simulink model "TB07_Integrated_Charging"  (R2025a)
settings: Solver=FixedStepDiscrete  StartTime=0  StopTime=TB.t_end  FixedStep=TB.dt  RelTol=1e-3
InitFcn:
  | % 모델과 같은 폴더의 초기화 스크립트를 실행해 P(설계 파라미터)와 TB(시험 조건)를 만든다.
  | run(fullfile(fileparts(get_param(bdroot, 'FileName')), 'TB07_init.m'));
values from neighbouring files (symbols this model uses):
  TB = struct()    [TB07_init.m]
libraries: fl_lib x207, nesl_utility x86
(part 1 of 5)
settings Model: Creator=hj000  LastModifiedBy=hj000
settings DataIOCC: SaveOutput=off  SignalLogging=off  SaveTime=off

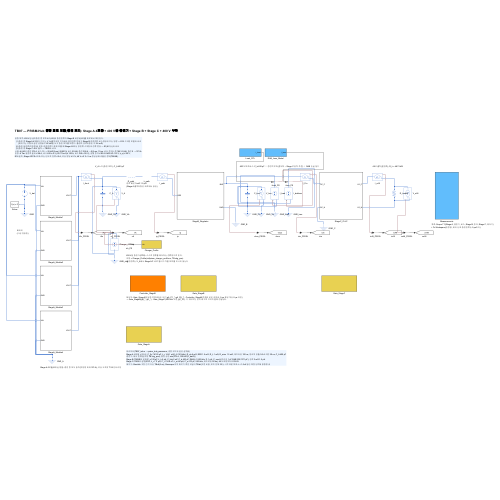
[thumbnail: Simulink's stored preview of the top-level diagram]
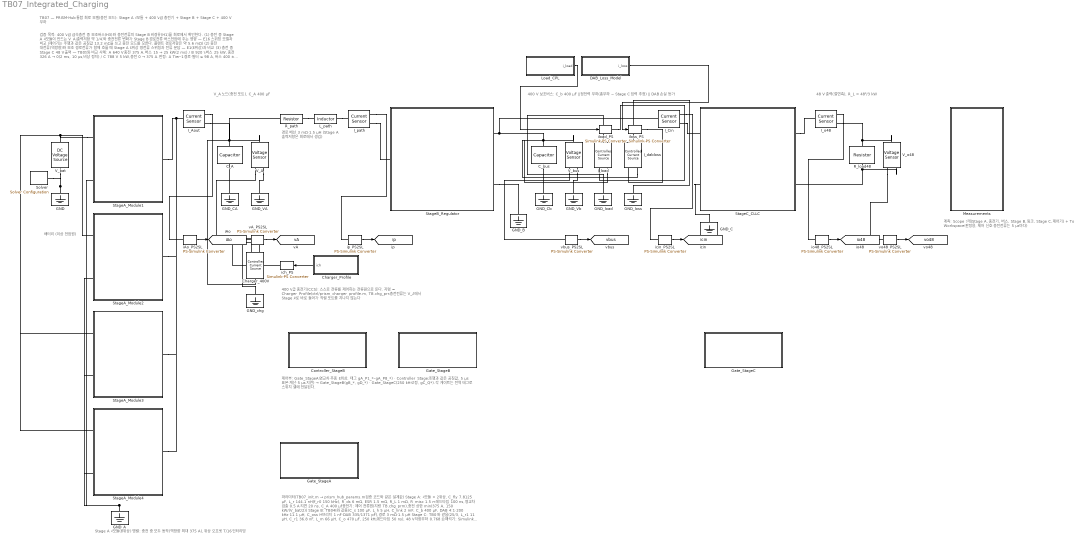
== system TB07_Integrated_Charging ==
  note: TB07 — PRISM-Hub 통합 회로 모델(충전 모드): Stage A 4모듈 + 400 V급 충전기 + Stage B + Stage C + 400 V 부하
  note: 검증 목적: 400 V급 급속충전 중 보조버스(H3)와 충전전류의 Stage B 비경유(H1)를 회로에서 확인한다.
      |   (1) 충전 중 Stage A 4모듈이 만드는 V_A(출력저항 약 1/4)와 충전전류 변화가 Stage B 경로전류·버스전압에 주는 영향 — E16 스위칭 모델과 비교
      |       (제어기는 주행과 같은 공칭값 13.2 mΩ을 쓰고 충전 모드를 모른다. 플랜트 경로저항은 약 5.6 mΩ)
      |   (2) 충전 대전류(역방향)와 보조 경로전류가 함께 흐를 때 Stage A 8위상 영전류 스위칭과 전류 분담 — E1(8위상)과 비교
      |   (3) 충전 중 Stage C 48 V 출력 — TB05와 비교
      | 사례: A 640 V 충전 375 A, 버스 15 → 25 kW(2 ms) / B 920 V 버스 25 kW, 충전 326 A → 0(2 ms, 10 µs, 비상 정지) / C 788 V 5 kW, 충전 0 → 375 A.
      | 판정: A Tier-1(경로·필터 ≤ 98 A, 버스 400 ± 8 V), B·C Tier-2(≤ 100 A, 버스 384–416 V), 공통 링크 ≤ 80 A·8 kW·90–110 V, |v_s| ≤ 90 V,
      | E16 일치, Stage A ZCS ≤ 5 % 또는 턴오프 전류 ≤ 2 A, 위상 분담 ≤ 5 %, 48 V ± 2 %. 5 ns 정상상태 리플은 정보(TB04B).
  note: 배터리
      | (이상 전압원)
  note: V_A 노드(충전 포트), C_A 400 µF
  note: 400 V급 충전기(CCS): 스스로 전류를 제어하는 전류원으로 둔다.
      | 지령 = Charger_Profile(ctrl/prism_charger_profile.m, TB.chg_prm)
      | 충전전류는 V_A에서 Stage A로 바로 들어가 직렬 포트를 지나지 않는다
  note: Stage A 4모듈(8위상) 병렬: 충전 중 모두 동작(역방향 최대 375 A), 위상 오프셋 T/16 인터리빙
  note: 경로 배선 3 mΩ·1.5 µH
      | (Stage A 출력저항은 회로에서 생김)
  note: 400 V 보조버스: C_b 400 µF ∥ 정전력 부하(총부하 − Stage C 입력 추정) ∥ DAB 손실 등가
  note: 48 V 출력(절연측), R_L = 48²/3 kW
  note: 제어부: Gate_StageA(영교차 추종 8위상, 태그 gA_P1_*–gA_P8_*) · Controller_StageB(주행과 같은 공칭값, 5 µs 표본·계산·5 µs 지연)
      | → Gate_StageB(gB_*, gD_*) · Gate_StageC(250 kHz 고정, gC_Q*). 각 게이트는 전역 태그로 스위치 셀에 전달된다.
  note: 계측: Scope 7개(Stage A, 충전기, 버스, Stage B, 링크, Stage C, 제어기)
      | + To Workspace(판정용, 제어 신호·충전전류는 5 µs마다)
  note: 파라미터(TB07_init.m → prism_hub_params.m, 검증 코드와 같은 설계값)
      | Stage A: 4모듈 × 2위상, C_fly 7.8125 µF, L_r 144.1 nH(f_r0 150 kHz), R_ds 6 mΩ, ESR 1.5 mΩ, R_L 1 mΩ, R_misc 1.5 mΩ, 데드타임 100 ns, 영교차 검출 0.5 A·지연 20 ns, C_A 400 µF
      | 충전기: 제어 전류원(지령 TB.chg_prm), 충전 상한 min(375 A, 150 kW/(V_bat/2))
      | Stage B: TB04B와 같음(C_s 100 µF, L_h 5 µH, C_link 2 mF, C_b 400 µF, DAB 4:1·200 kHz·11.1 µH, C_oss H-브리지 1 nF·DAB 335/1371 pF), 경로 3 mΩ·1.5 µH
      | Stage C: TB05와 같음(25/3, L_r1 11 µH, C_r1 36.8 nF, L_m 66 µH, C_o 470 µF, 250 kHz, 데드타임 50 ns), 48 V 저항부하 0.768 Ω
      | 해석기: Simulink 고정 간격 이산 TB.dt(5 ns), Simscape 지역 해석기 후진 오일러 TB.dt(고정 비용, 모드 반복 3회). 시작 표본 보호: t < 1.5 dt 동안 측정 입력에 평형점 값
  C_A : fl_lib/Electrical/Electrical Elements/Capacitor  c=TB.A.CA F  r=1e-6 Ohm  g=0 1/Ohm  i_specify=off  i_priority=None  i=0 A  i_nominal_specify=off  i_nominal_value=1  i_nominal_unit=A  v_specify=off  v_priority=None  v=0 V  v_nominal_specify=off  v_nominal_value=1  v_nominal_unit=V  vc_specify=on  vc_priority=High  vc=TB.vA0 V  vc_nominal_specify=off  vc_nominal_value=1  vc_nominal_unit=V
  C_bus : fl_lib/Electrical/Electrical Elements/Capacitor  c=TB.Cb F  r=1e-6 Ohm  g=0 1/Ohm  i_specify=off  i_priority=None  i=0 A  i_nominal_specify=off  i_nominal_value=1  i_nominal_unit=A  v_specify=off  v_priority=None  v=0 V  v_nominal_specify=off  v_nominal_value=1  v_nominal_unit=V  vc_specify=on  vc_priority=High  vc=TB.vb0 V  vc_nominal_specify=off  vc_nominal_value=1  vc_nominal_unit=V
  Charger_400V : fl_lib/Electrical/Electrical Sources/Controlled Current Source
  Charger_Profile : Subsystem
  Controller_StageB : Subsystem
  DAB_Loss_Model : Subsystem
  GND : fl_lib/Electrical/Electrical Elements/Electrical Reference
  GND_A : fl_lib/Electrical/Electrical Elements/Electrical Reference
  GND_B : fl_lib/Electrical/Electrical Elements/Electrical Reference
  GND_C : fl_lib/Electrical/Electrical Elements/Electrical Reference
  GND_CA : fl_lib/Electrical/Electrical Elements/Electrical Reference
  GND_Cb : fl_lib/Electrical/Electrical Elements/Electrical Reference
  GND_VA : fl_lib/Electrical/Electrical Elements/Electrical Reference
  GND_Vb : fl_lib/Electrical/Electrical Elements/Electrical Reference
  GND_chg : fl_lib/Electrical/Electrical Elements/Electrical Reference
  GND_load : fl_lib/Electrical/Electrical Elements/Electrical Reference
  GND_loss : fl_lib/Electrical/Electrical Elements/Electrical Reference
  Gate_StageA : Subsystem
  Gate_StageB : Subsystem
  Gate_StageC : Subsystem
  I_Aout : fl_lib/Electrical/Electrical Sensors/Current Sensor
  I_Cin : fl_lib/Electrical/Electrical Sensors/Current Sensor
  I_dabloss : fl_lib/Electrical/Electrical Sources/Controlled Current Source
  I_load : fl_lib/Electrical/Electrical Sources/Controlled Current Source
  I_o48 : fl_lib/Electrical/Electrical Sensors/Current Sensor
  I_path : fl_lib/Electrical/Electrical Sensors/Current Sensor
  L_path : fl_lib/Electrical/Electrical Elements/Inductor  l=TB.Lpath H  r=0 Ohm  g=1e-9 1/Ohm  i_specify=off  i_priority=None  i=0 A  i_nominal_specify=off  i_nominal_value=1  i_nominal_unit=A  v_specify=off  v_priority=None  v=0 V  v_nominal_specify=off  v_nominal_value=1  v_nominal_unit=V  i_L_specify=on  i_L_priority=High  i_L=TB.ip0 A  i_L_nominal_specify=off  i_L_nominal_value=1  i_L_nominal_unit=A
  Load_CPL : Subsystem
  Measurements : Subsystem
  R_load48 : fl_lib/Electrical/Electrical Elements/Resistor  R=TB.RL_C Ohm  i_specify=off  i_priority=None  i=0 A  i_nominal_specify=off  i_nominal_value=1  i_nominal_unit=A  v_specify=off  v_priority=None  v=0 V  v_nominal_specify=off  v_nominal_value=1  v_nominal_unit=V
  R_path : fl_lib/Electrical/Electrical Elements/Resistor  R=TB.Rpath Ohm  i_specify=off  i_priority=None  i=0 A  i_nominal_specify=off  i_nominal_value=1  i_nominal_unit=A  v_specify=off  v_priority=None  v=0 V  v_nominal_specify=off  v_nominal_value=1  v_nominal_unit=V
  Solver : nesl_utility/Solver Configuration  PhysicalDomain=network_engine_domain  SubClassName=solver  LeftPortType=input  RightPortType=generic  Tones=[]  Harmonics=[]  SimulateNoise=off  Profile=off  UseLocalSampling=off  EnableSwitchedLinearOptims=on  FrequencyDomain=off  UseCCode=off  RelTol=0.001  AbsTol=0.001  MinStep=1e-09  ToWorkspace=off  RevertToSquareIcSolve=off  NumHomotopyIterations=100  PhasorMode=off  PhasorModeNumHarmonics=1  ConsistencySolver=NEWTON_XTOL_AFTER_FTOL  IndexReductionMethod=DerivativeReplacement  DoDC=off  ResidualTolerance=1e-9  ConsistencyTolSource=GLOBAL  ConsistencyAbsTol=0.001  ConsistencyRelTol=0.001  ConsistencyTolFactor=0.001  UseLocalSolver=on  LocalSolverChoice=NE_BACKWARD_EULER_ADVANCER  ResolveIndetEquations=on  FunctionEvalNumThread=1  LocalSolverSampleTime=TB.dt  DoFixedCost=on  MaxNonlinIter=3  MaxModeIter=2  ComputeImpulses=off  ImpulseIterations=2  LinearAlgebra=auto  LinearAlgebraNumThread=0  EquationFormulation=NE_TIME_EF  DelaysMemoryBudget=1024  AutomaticFiltering=on  FilteringTimeConstant=0.001  PartitionStorageMethod=AS_NEEDED  PartitionMemoryBudget=1024  PartitionMethod=ROBUST  MultibodyUseLocalSolver=off  MultibodyLocalSolverChoice=ODE1  MultibodyLocalSolverSampleTime=0.001
  StageA_Module1 : Subsystem
  StageA_Module2 : Subsystem
  StageA_Module3 : Subsystem
  StageA_Module4 : Subsystem
  StageB_Regulator : Subsystem
  StageC_CLLC : Subsystem
  V_A : fl_lib/Electrical/Electrical Sensors/Voltage Sensor
  V_bat : fl_lib/Electrical/Electrical Sources/DC Voltage Source  v0=TB.vbat V
  V_bus : fl_lib/Electrical/Electrical Sensors/Voltage Sensor
  V_o48 : fl_lib/Electrical/Electrical Sensors/Voltage Sensor
  iAo_PS2SL : nesl_utility/PS-Simulink Converter  PhysicalDomain=network_engine_domain  SubClassName=ps_output  LeftPortType=input  RightPortType=output  PseudoPeriodic=off  Frequencies=[]  VectorFormat=inherit  Unit=inherit  AffineConversion=off
  ich_PS : nesl_utility/Simulink-PS Converter  PhysicalDomain=network_engine_domain  SubClassName=ps_input  LeftPortType=input  RightPortType=output  PseudoPeriodic=off  Frequencies=[]  NoiseDistribution=none  NoiseParameters=[]  Unit=1  AffineConversion=off  FilteringAndDerivatives=provide  SimscapeFilterOrder=1  InputFilterTimeConstant=0.001  UdotUserProvided=0
  icin_PS2SL : nesl_utility/PS-Simulink Converter  PhysicalDomain=network_engine_domain  SubClassName=ps_output  LeftPortType=input  RightPortType=output  PseudoPeriodic=off  Frequencies=[]  VectorFormat=inherit  Unit=inherit  AffineConversion=off
  iload_PS : nesl_utility/Simulink-PS Converter  PhysicalDomain=network_engine_domain  SubClassName=ps_input  LeftPortType=input  RightPortType=output  PseudoPeriodic=off  Frequencies=[]  NoiseDistribution=none  NoiseParameters=[]  Unit=1  AffineConversion=off  FilteringAndDerivatives=provide  SimscapeFilterOrder=1  InputFilterTimeConstant=0.001  UdotUserProvided=0
  iloss_PS : nesl_utility/Simulink-PS Converter  PhysicalDomain=network_engine_domain  SubClassName=ps_input  LeftPortType=input  RightPortType=output  PseudoPeriodic=off  Frequencies=[]  NoiseDistribution=none  NoiseParameters=[]  Unit=1  AffineConversion=off  FilteringAndDerivatives=provide  SimscapeFilterOrder=1  InputFilterTimeConstant=0.001  UdotUserProvided=0
  io48_PS2SL : nesl_utility/PS-Simulink Converter  PhysicalDomain=network_engine_domain  SubClassName=ps_output  LeftPortType=input  RightPortType=output  PseudoPeriodic=off  Frequencies=[]  VectorFormat=inherit  Unit=inherit  AffineConversion=off
  ip_PS2SL : nesl_utility/PS-Simulink Converter  PhysicalDomain=network_engine_domain  SubClassName=ps_output  LeftPortType=input  RightPortType=output  PseudoPeriodic=off  Frequencies=[]  VectorFormat=inherit  Unit=inherit  AffineConversion=off
  vA_PS2SL : nesl_utility/PS-Simulink Converter  PhysicalDomain=network_engine_domain  SubClassName=ps_output  LeftPortType=input  RightPortType=output  PseudoPeriodic=off  Frequencies=[]  VectorFormat=inherit  Unit=inherit  AffineConversion=off
  vbus_PS2SL : nesl_utility/PS-Simulink Converter  PhysicalDomain=network_engine_domain  SubClassName=ps_output  LeftPortType=input  RightPortType=output  PseudoPeriodic=off  Frequencies=[]  VectorFormat=inherit  Unit=inherit  AffineConversion=off
  vo48_PS2SL : nesl_utility/PS-Simulink Converter  PhysicalDomain=network_engine_domain  SubClassName=ps_output  LeftPortType=input  RightPortType=output  PseudoPeriodic=off  Frequencies=[]  VectorFormat=inherit  Unit=inherit  AffineConversion=off
  tag scope: iAo=global, icin=global, io48=global, ip=global, vA=global, vbus=global, vo48=global
  wires:
  iAo_PS2SL/1 -> [iAo]
  vA_PS2SL/1 -> [vA]
  ip_PS2SL/1 -> [ip]
  vbus_PS2SL/1 -> [vbus]
  icin_PS2SL/1 -> [icin]
  io48_PS2SL/1 -> [io48]
  vo48_PS2SL/1 -> [vo48]
  Load_CPL/1(i_load) -> iload_PS/1
  DAB_Loss_Model/1(i_loss) -> iloss_PS/1
  Charger_Profile/1(ich) -> ich_PS/1
  connections:
  GND/LConn1 -- Solver/RConn1 -- V_bat/RConn1
  StageA_Module1/LConn1 -- V_bat/LConn1 -- StageA_Module2/LConn1 -- StageA_Module3/LConn1 -- StageA_Module4/LConn1
  StageA_Module1/LConn2 -- StageA_Module2/LConn2 -- StageA_Module3/LConn2 -- GND_A/LConn1 -- StageA_Module4/LConn2
  StageA_Module1/RConn1 -- StageA_Module2/RConn1 -- StageA_Module3/RConn1 -- I_Aout/LConn1 -- StageA_Module4/RConn1
  I_Aout/RConn2 -- V_A/LConn1 -- Charger_400V/LConn1 -- C_A/LConn1 -- R_path/LConn1
  C_A/RConn1 -- GND_CA/LConn1
  V_A/RConn2 -- GND_VA/LConn1
  Charger_400V/RConn2 -- GND_chg/LConn1
  ich_PS/RConn1 -- Charger_400V/RConn1
  R_path/RConn1 -- L_path/LConn1
  L_path/RConn1 -- I_path/LConn1
  I_path/RConn2 -- StageB_Regulator/LConn1
  StageB_Regulator/RConn1 -- I_Cin/LConn1 -- V_bus/LConn1 -- I_load/RConn2 -- C_bus/LConn1 -- I_dabloss/RConn2
  StageB_Regulator/RConn2 -- GND_B/LConn1
  C_bus/RConn1 -- GND_Cb/LConn1
  V_bus/RConn2 -- GND_Vb/LConn1
  I_load/LConn1 -- GND_load/LConn1
  I_dabloss/LConn1 -- GND_loss/LConn1
  iload_PS/RConn1 -- I_load/RConn1
  iloss_PS/RConn1 -- I_dabloss/RConn1
  I_Cin/RConn2 -- StageC_CLLC/LConn1
  StageC_CLLC/LConn2 -- GND_C/LConn1
  StageC_CLLC/RConn1 -- I_o48/LConn1
  R_load48/LConn1 -- I_o48/RConn2 -- V_o48/LConn1
  StageC_CLLC/RConn2 -- R_load48/RConn1 -- V_o48/RConn2
  I_Aout/RConn1 -- iAo_PS2SL/LConn1
  V_A/RConn1 -- vA_PS2SL/LConn1
  I_path/RConn1 -- ip_PS2SL/LConn1
  V_bus/RConn1 -- vbus_PS2SL/LConn1
  I_Cin/RConn1 -- icin_PS2SL/LConn1
  I_o48/RConn1 -- io48_PS2SL/LConn1
  V_o48/RConn1 -- vo48_PS2SL/LConn1

== system TB07_Integrated_Charging/Charger_Profile ==
  note: 충전기 출력전류 지령 [i0 i1 t_sw t_ramp]: t_sw부터 t_ramp 동안 i0 → i1 선형
  Charger_Current : MATLAB Function  TreatAsAtomicUnit=on
  Clock : DigitalClock  SampleTime=TB.dt
  chg_prm : Constant  Value=TB.chg_prm
  ich : Outport
  tag scope: ich=global
  wires:
  Clock/1 -> Charger_Current/1(t)
  chg_prm/1 -> Charger_Current/2(prm)
  Charger_Current/1(ich) -> ich/1, [ich]

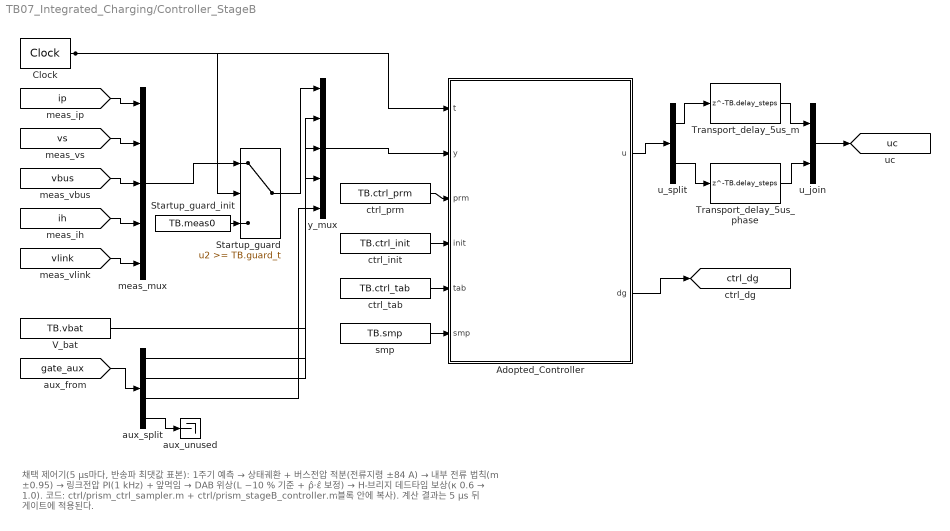
== system TB07_Integrated_Charging/Controller_StageB ==
  note: 채택 제어기(5 µs마다, 반송파 최댓값 표본): 1주기 예측 → 상태궤환 + 버스전압 적분(전류지령 ±84 A) → 내부 전류 법칙(m ±0.95)
      | → 링크전압 PI(1 kHz) + 앞먹임 → DAB 위상(L −10 % 기준 + ρ̂·ε̂ 보정) → H-브리지 데드타임 보상(κ 0.6 → 1.0).
      | 코드: ctrl/prism_ctrl_sampler.m + ctrl/prism_stageB_controller.m(블록 안에 복사). 계산 결과는 5 µs 뒤 게이트에 적용된다.
  Adopted_Controller : MATLAB Function  TreatAsAtomicUnit=on
  Clock : DigitalClock  SampleTime=TB.dt
  Startup_guard : Switch  Threshold=TB.guard_t  SaturateOnIntegerOverflow=off  InputSameDT=off
  Startup_guard_init : Constant  Value=TB.meas0
  Transport_delay_5us_m : Delay  DelayLength=TB.delay_steps  InitialCondition=TB.uc0(1)
  Transport_delay_5us_phase : Delay  DelayLength=TB.delay_steps  InitialCondition=TB.uc0(2)
  V_bat : Constant  Value=TB.vbat
  aux_split : Demux  Outputs=[1 1 1 3]
  aux_unused : Terminator
  ctrl_init : Constant  Value=TB.ctrl_init
  ctrl_prm : Constant  Value=TB.ctrl_prm
  ctrl_tab : Constant  Value=TB.ctrl_tab
  meas_mux : Mux  Inputs=5
  smp : Constant  Value=TB.smp
  u_join : Mux  Inputs=2
  u_split : Demux  Outputs=2
  y_mux : Mux  Inputs=5
  tag scope: ctrl_dg=global, uc=global
  wires:
  [ip] -> meas_mux/1
  [vs] -> meas_mux/2
  [vbus] -> meas_mux/3
  [ih] -> meas_mux/4
  [vlink] -> meas_mux/5
  Startup_guard_init/1 -> Startup_guard/3
  meas_mux/1 -> Startup_guard/1
  Clock/1 -> Startup_guard/2, Adopted_Controller/1(t)
  Startup_guard/1 -> y_mux/1
  V_bat/1 -> y_mux/2
  [gate_aux] -> aux_split/1
  aux_split/1 -> y_mux/3
  aux_split/2 -> y_mux/4
  aux_split/3 -> y_mux/5
  aux_split/4 -> aux_unused/1
  y_mux/1 -> Adopted_Controller/2(y)
  ctrl_prm/1 -> Adopted_Controller/3(prm)
  ctrl_init/1 -> Adopted_Controller/4(init)
  ctrl_tab/1 -> Adopted_Controller/5(tab)
  smp/1 -> Adopted_Controller/6(smp)
  Adopted_Controller/1(u) -> u_split/1
  u_split/1 -> Transport_delay_5us_m/1
  u_split/2 -> Transport_delay_5us_phase/1
  Transport_delay_5us_m/1 -> u_join/1
  Transport_delay_5us_phase/1 -> u_join/2
  u_join/1 -> [uc]
  Adopted_Controller/2(dg) -> [ctrl_dg]

== system TB07_Integrated_Charging/DAB_Loss_Model ==
  note: DAB 손실 등가: 직전 주기 평균 링크전력 p̄로 P_loss = (1/η − 1)max(p̄,0) + (1 − η)max(−p̄,0) − R_dab·mean(i_L²)
      | (η = 0.96, 검증 모델과 같음)을 버스 전류 P_loss/v_bus로 끈다. 회로의 R_dab 손실은 빼서 중복을 막는다.
  Clock : DigitalClock  SampleTime=TB.dt
  DAB_Loss : MATLAB Function  TreatAsAtomicUnit=on
  Startup_guard : Switch  Threshold=TB.guard_t  SaturateOnIntegerOverflow=off  InputSameDT=off
  Startup_guard_init : Constant  Value=TB.loss_meas0
  iloss_z1 : UnitDelay  SampleTime=TB.dt  HasFrameUpgradeWarning=on
  loss_prm : Constant  Value=TB.loss_prm
  meas_mux : Mux
  meas_split : Demux
  ploss0 : Constant  Value=TB.ploss0
  i_loss : Outport
  wires:
  [vlink] -> meas_mux/1
  [ilink] -> meas_mux/2
  [iL] -> meas_mux/3
  [vbus] -> meas_mux/4
  Startup_guard_init/1 -> Startup_guard/3
  meas_mux/1 -> Startup_guard/1
  Clock/1 -> Startup_guard/2, DAB_Loss/1(t)
  Startup_guard/1 -> meas_split/1
  meas_split/1 -> DAB_Loss/2(vl)
  meas_split/2 -> DAB_Loss/3(il)
  meas_split/3 -> DAB_Loss/4(iL)
  meas_split/4 -> DAB_Loss/5(vb)
  loss_prm/1 -> DAB_Loss/6(prm)
  ploss0/1 -> DAB_Loss/7(ploss0)
  DAB_Loss/1(iloss) -> iloss_z1/1
  iloss_z1/1 -> i_loss/1

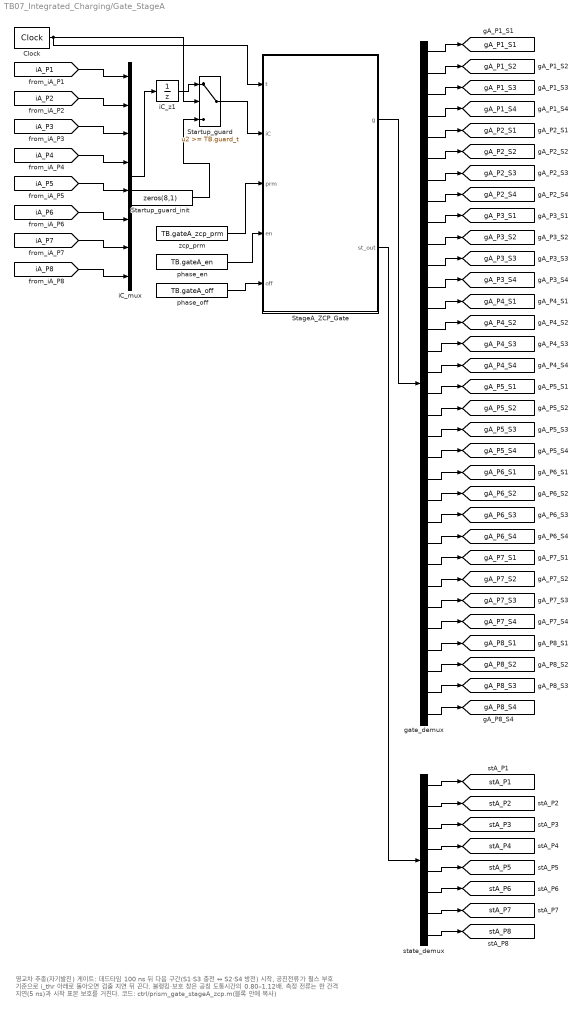
== system TB07_Integrated_Charging/Gate_StageA ==
  note: 영교차 추종(자기발진) 게이트: 데드타임 100 ns 뒤 다음 구간(S1·S3 충전 ↔ S2·S4 방전) 시작,
      | 공진전류가 펄스 부호 기준으로 i_thr 아래로 돌아오면 검출 지연 뒤 끈다. 블랭킹·보호 창은 공칭 도통시간의 0.80–1.12배.
      | 측정 전류는 한 간격 지연(5 ns)과 시작 표본 보호를 거친다. 코드: ctrl/prism_gate_stageA_zcp.m(블록 안에 복사)
  Clock : DigitalClock  SampleTime=TB.dt
  StageA_ZCP_Gate : MATLAB Function  TreatAsAtomicUnit=on
  Startup_guard : Switch  Threshold=TB.guard_t  SaturateOnIntegerOverflow=off  InputSameDT=off
  Startup_guard_init : Constant  Value=zeros(8,1)
  gate_demux : Demux  Outputs=[1 1 1 1 1 1 1 1 1 1 1 1 1 1 1 1 1 1 1 1 1 1 1 1 1 1 1 1 1 1 1 1]
  iC_mux : Mux  Inputs=8
  iC_z1 : UnitDelay  SampleTime=TB.dt  HasFrameUpgradeWarning=on
  phase_en : Constant  Value=TB.gateA_en
  phase_off : Constant  Value=TB.gateA_off
  state_demux : Demux  Outputs=[1 1 1 1 1 1 1 1]
  zcp_prm : Constant  Value=TB.gateA_zcp_prm
  tag scope: gA_P1_S1=global, gA_P1_S2=global, gA_P1_S3=global, gA_P1_S4=global, gA_P2_S1=global, gA_P2_S2=global, gA_P2_S3=global, gA_P2_S4=global, gA_P3_S1=global, gA_P3_S2=global, gA_P3_S3=global, gA_P3_S4=global, gA_P4_S1=global, gA_P4_S2=global, gA_P4_S3=global, gA_P4_S4=global, gA_P5_S1=global, gA_P5_S2=global, gA_P5_S3=global, gA_P5_S4=global, gA_P6_S1=global, gA_P6_S2=global, gA_P6_S3=global, gA_P6_S4=global, gA_P7_S1=global, gA_P7_S2=global, gA_P7_S3=global, gA_P7_S4=global, gA_P8_S1=global, gA_P8_S2=global, gA_P8_S3=global, gA_P8_S4=global, stA_P1=global, stA_P2=global, stA_P3=global, stA_P4=global, stA_P5=global, stA_P6=global, stA_P7=global, stA_P8=global
  wires:
  [iA_P1] -> iC_mux/1
  [iA_P2] -> iC_mux/2
  [iA_P3] -> iC_mux/3
  [iA_P4] -> iC_mux/4
  [iA_P5] -> iC_mux/5
  [iA_P6] -> iC_mux/6
  [iA_P7] -> iC_mux/7
  [iA_P8] -> iC_mux/8
  iC_mux/1 -> iC_z1/1
  Startup_guard_init/1 -> Startup_guard/3
  iC_z1/1 -> Startup_guard/1
  Clock/1 -> Startup_guard/2, StageA_ZCP_Gate/1(t)
  Startup_guard/1 -> StageA_ZCP_Gate/2(iC)
  zcp_prm/1 -> StageA_ZCP_Gate/3(prm)
  phase_en/1 -> StageA_ZCP_Gate/4(en)
  phase_off/1 -> StageA_ZCP_Gate/5(off)
  StageA_ZCP_Gate/1(g) -> gate_demux/1
  gate_demux/1 -> [gA_P1_S1]
  gate_demux/2 -> [gA_P1_S2]
  gate_demux/3 -> [gA_P1_S3]
  gate_demux/4 -> [gA_P1_S4]
  gate_demux/5 -> [gA_P2_S1]
  gate_demux/6 -> [gA_P2_S2]
  gate_demux/7 -> [gA_P2_S3]
  gate_demux/8 -> [gA_P2_S4]
  gate_demux/9 -> [gA_P3_S1]
  gate_demux/10 -> [gA_P3_S2]
  gate_demux/11 -> [gA_P3_S3]
  gate_demux/12 -> [gA_P3_S4]
  gate_demux/13 -> [gA_P4_S1]
  gate_demux/14 -> [gA_P4_S2]
  gate_demux/15 -> [gA_P4_S3]
  gate_demux/16 -> [gA_P4_S4]
  gate_demux/17 -> [gA_P5_S1]
  gate_demux/18 -> [gA_P5_S2]
  gate_demux/19 -> [gA_P5_S3]
  gate_demux/20 -> [gA_P5_S4]
  gate_demux/21 -> [gA_P6_S1]
  gate_demux/22 -> [gA_P6_S2]
  gate_demux/23 -> [gA_P6_S3]
  gate_demux/24 -> [gA_P6_S4]
  gate_demux/25 -> [gA_P7_S1]
  gate_demux/26 -> [gA_P7_S2]
  gate_demux/27 -> [gA_P7_S3]
  gate_demux/28 -> [gA_P7_S4]
  gate_demux/29 -> [gA_P8_S1]
  gate_demux/30 -> [gA_P8_S2]
  gate_demux/31 -> [gA_P8_S3]
  gate_demux/32 -> [gA_P8_S4]
  StageA_ZCP_Gate/2(st_out) -> state_demux/1
  state_demux/1 -> [stA_P1]
  state_demux/2 -> [stA_P2]
  state_demux/3 -> [stA_P3]
  state_demux/4 -> [stA_P4]
  state_demux/5 -> [stA_P5]
  state_demux/6 -> [stA_P6]
  state_demux/7 -> [stA_P7]
  state_demux/8 -> [stA_P8]

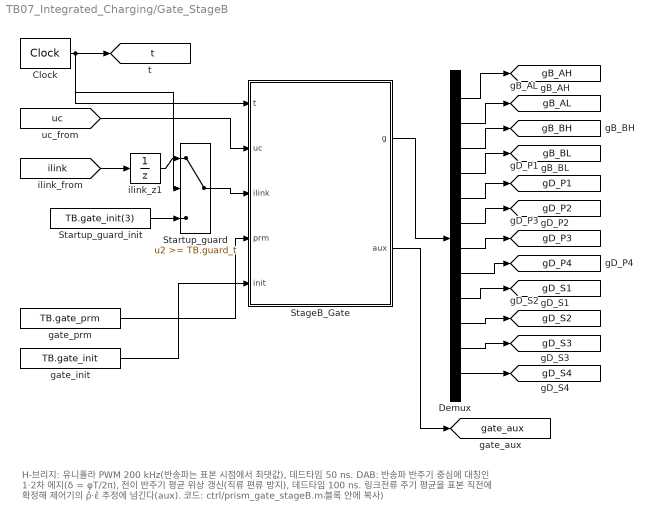
== system TB07_Integrated_Charging/Gate_StageB ==
  note: H-브리지: 유니폴라 PWM 200 kHz(반송파는 표본 시점에서 최댓값), 데드타임 50 ns.
      | DAB: 반송파 반주기 중심에 대칭인 1·2차 에지(δ = φT/2π), 전이 반주기 평균 위상 갱신(직류 편류 방지), 데드타임 100 ns.
      | 링크전류 주기 평균을 표본 직전에 확정해 제어기의 ρ̂·ε̂ 추정에 넘긴다(aux). 코드: ctrl/prism_gate_stageB.m(블록 안에 복사)
  Clock : DigitalClock  SampleTime=TB.dt
  Demux : Demux  Outputs=12
  StageB_Gate : MATLAB Function  TreatAsAtomicUnit=on
  Startup_guard : Switch  Threshold=TB.guard_t  SaturateOnIntegerOverflow=off  InputSameDT=off
  Startup_guard_init : Constant  Value=TB.gate_init(3)
  gate_init : Constant  Value=TB.gate_init
  gate_prm : Constant  Value=TB.gate_prm
  ilink_z1 : UnitDelay  SampleTime=TB.dt  HasFrameUpgradeWarning=on
  tag scope: gB_AH=global, gB_AL=global, gB_BH=global, gB_BL=global, gD_P1=global, gD_P2=global, gD_P3=global, gD_P4=global, gD_S1=global, gD_S2=global, gD_S3=global, gD_S4=global, gate_aux=global, t=global
  wires:
  Startup_guard_init/1 -> Startup_guard/3
  Clock/1 -> [t], StageB_Gate/1(t), Startup_guard/2
  [uc] -> StageB_Gate/2(uc)
  [ilink] -> ilink_z1/1
  ilink_z1/1 -> Startup_guard/1
  Startup_guard/1 -> StageB_Gate/3(ilink)
  gate_prm/1 -> StageB_Gate/4(prm)
  gate_init/1 -> StageB_Gate/5(init)
  StageB_Gate/1(g) -> Demux/1
  Demux/1 -> [gB_AH]
  Demux/2 -> [gB_AL]
  Demux/3 -> [gB_BH]
  Demux/4 -> [gB_BL]
  Demux/5 -> [gD_P1]
  Demux/6 -> [gD_P2]
  Demux/7 -> [gD_P3]
  Demux/8 -> [gD_P4]
  Demux/9 -> [gD_S1]
  Demux/10 -> [gD_S2]
  Demux/11 -> [gD_S3]
  Demux/12 -> [gD_S4]
  StageB_Gate/2(aux) -> [gate_aux]

== system TB07_Integrated_Charging/Gate_StageC ==
  note: Stage C 게이트: 주기 T = 4 µs(공진점 250 kHz), 전반주기 [t_d, T/2) Q1·Q4, 후반주기 [T/2 + t_d, T) Q2·Q3, 데드타임 50 ns.
      | 고정이득 구조이므로 폐루프 제어는 없다(48 V는 Stage B가 조정한 400 V 버스에서 간접적으로 정해진다).
  Clock : DigitalClock  SampleTime=TB.dt
  Demux : Demux
  StageC_Gate : MATLAB Function  TreatAsAtomicUnit=on
  gate_prm : Constant  Value=TB.gateC_prm
  tag scope: gC_Q1=global, gC_Q2=global, gC_Q3=global, gC_Q4=global
  wires:
  Clock/1 -> StageC_Gate/1(t)
  gate_prm/1 -> StageC_Gate/2(prm)
  StageC_Gate/1(g) -> Demux/1
  Demux/1 -> [gC_Q1]
  Demux/2 -> [gC_Q2]
  Demux/3 -> [gC_Q3]
  Demux/4 -> [gC_Q4]

== system TB07_Integrated_Charging/Load_CPL ==
  note: 정전력 부하: i = P(t)/max(v_bus, v_min). v_bus는 시작 표본 보호 후 한 간격 지연
  P_over_v : Product  Inputs=*/
  P_profile : Step  Time=TB.t_step  Before=TB.P0  After=TB.P1  SampleTime=TB.dt
  Startup_guard : Switch  Threshold=TB.guard_t  SaturateOnIntegerOverflow=off  InputSameDT=off
  Startup_guard_init : Constant  Value=TB.vb0
  v_floor : MinMax  Function=max  Inputs=2
  v_min : Constant  Value=TB.vmin
  vbus_z1 : UnitDelay  SampleTime=TB.dt  HasFrameUpgradeWarning=on
  i_load : Outport
  tag scope: p_load=global
  wires:
  Startup_guard_init/1 -> Startup_guard/3
  P_profile/1 -> [p_load], P_over_v/1
  [vbus] -> Startup_guard/1
  [t] -> Startup_guard/2
  Startup_guard/1 -> vbus_z1/1
  vbus_z1/1 -> v_floor/1
  v_min/1 -> v_floor/2
  v_floor/1 -> P_over_v/2
  P_over_v/1 -> i_load/1

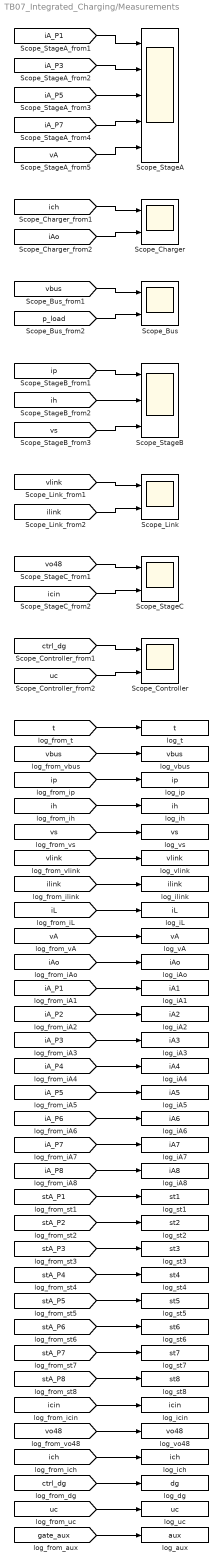
== system TB07_Integrated_Charging/Measurements ==
  Scope_Bus : Scope  NumInputPorts=2
      settings: Title=Scope Bus
  Scope_Charger : Scope  NumInputPorts=2
      settings: Title=Scope Charger
  Scope_Controller : Scope  NumInputPorts=2
      settings: Title=Scope Controller
  Scope_Link : Scope  NumInputPorts=2
      settings: Title=Scope Link
  Scope_StageA : Scope  NumInputPorts=5
      settings: Title=Scope StageA
  Scope_StageB : Scope  NumInputPorts=3
      settings: Title=Scope StageB
  Scope_StageC : Scope  NumInputPorts=2
      settings: Title=Scope StageC
  log_aux : ToWorkspace  VariableName=aux  SampleTime=-1
      settings: Decimation=TB.Np
  log_dg : ToWorkspace  VariableName=dg  SampleTime=-1
      settings: Decimation=TB.Np
  log_iA1 : ToWorkspace  VariableName=iA1  SampleTime=-1
  log_iA2 : ToWorkspace  VariableName=iA2  SampleTime=-1
  log_iA3 : ToWorkspace  VariableName=iA3  SampleTime=-1
  log_iA4 : ToWorkspace  VariableName=iA4  SampleTime=-1
  log_iA5 : ToWorkspace  VariableName=iA5  SampleTime=-1
  log_iA6 : ToWorkspace  VariableName=iA6  SampleTime=-1
  log_iA7 : ToWorkspace  VariableName=iA7  SampleTime=-1
  log_iA8 : ToWorkspace  VariableName=iA8  SampleTime=-1
  log_iAo : ToWorkspace  VariableName=iAo  SampleTime=-1
  log_iL : ToWorkspace  VariableName=iL  SampleTime=-1
  log_ich : ToWorkspace  VariableName=ich  SampleTime=-1
      settings: Decimation=TB.Np
  log_icin : ToWorkspace  VariableName=icin  SampleTime=-1
  log_ih : ToWorkspace  VariableName=ih  SampleTime=-1
  log_ilink : ToWorkspace  VariableName=ilink  SampleTime=-1
  log_ip : ToWorkspace  VariableName=ip  SampleTime=-1
  log_st1 : ToWorkspace  VariableName=st1  SampleTime=-1
  log_st2 : ToWorkspace  VariableName=st2  SampleTime=-1
  log_st3 : ToWorkspace  VariableName=st3  SampleTime=-1
  log_st4 : ToWorkspace  VariableName=st4  SampleTime=-1
  log_st5 : ToWorkspace  VariableName=st5  SampleTime=-1
  log_st6 : ToWorkspace  VariableName=st6  SampleTime=-1
  log_st7 : ToWorkspace  VariableName=st7  SampleTime=-1
  log_st8 : ToWorkspace  VariableName=st8  SampleTime=-1
  log_t : ToWorkspace  VariableName=t  SampleTime=-1
  log_uc : ToWorkspace  VariableName=uc  SampleTime=-1
      settings: Decimation=TB.Np
  log_vA : ToWorkspace  VariableName=vA  SampleTime=-1
  log_vbus : ToWorkspace  VariableName=vbus  SampleTime=-1
  log_vlink : ToWorkspace  VariableName=vlink  SampleTime=-1
  log_vo48 : ToWorkspace  VariableName=vo48  SampleTime=-1
  log_vs : ToWorkspace  VariableName=vs  SampleTime=-1
  wires:
  [iA_P1] -> Scope_StageA/1
  [iA_P3] -> Scope_StageA/2
  [iA_P5] -> Scope_StageA/3
  [iA_P7] -> Scope_StageA/4
  [vA] -> Scope_StageA/5
  [ich] -> Scope_Charger/1
  [iAo] -> Scope_Charger/2
  [vbus] -> Scope_Bus/1
  [p_load] -> Scope_Bus/2
  [ip] -> Scope_StageB/1
  [ih] -> Scope_StageB/2
  [vs] -> Scope_StageB/3
  [vlink] -> Scope_Link/1
  [ilink] -> Scope_Link/2
  [vo48] -> Scope_StageC/1
  [icin] -> Scope_StageC/2
  [ctrl_dg] -> Scope_Controller/1
  [uc] -> Scope_Controller/2
  [t] -> log_t/1
  [vbus] -> log_vbus/1
  [ip] -> log_ip/1
  [ih] -> log_ih/1
  [vs] -> log_vs/1
  [vlink] -> log_vlink/1
  [ilink] -> log_ilink/1
  [iL] -> log_iL/1
  [vA] -> log_vA/1
  [iAo] -> log_iAo/1
  [iA_P1] -> log_iA1/1
  [iA_P2] -> log_iA2/1
  [iA_P3] -> log_iA3/1
  [iA_P4] -> log_iA4/1
  [iA_P5] -> log_iA5/1
  [iA_P6] -> log_iA6/1
  [iA_P7] -> log_iA7/1
  [iA_P8] -> log_iA8/1
  [stA_P1] -> log_st1/1
  [stA_P2] -> log_st2/1
  [stA_P3] -> log_st3/1
  [stA_P4] -> log_st4/1
  [stA_P5] -> log_st5/1
  [stA_P6] -> log_st6/1
  [stA_P7] -> log_st7/1
  [stA_P8] -> log_st8/1
  [icin] -> log_icin/1
  [vo48] -> log_vo48/1
  [ich] -> log_ich/1
  [ctrl_dg] -> log_dg/1
  [uc] -> log_uc/1
  [gate_aux] -> log_aux/1

== system TB07_Integrated_Charging/StageA_Module1 ==
  note: Stage A 모듈 1: 위상 1·2 병렬(목표 정격 37.5 kW)
      | 각 위상은 영교차 추종 게이트로 자기 공진전류가 0일 때 끈다(ZCS). 두 위상은 T/4 엇갈려 시작한다.
  StageA_Phase1 : Subsystem
  StageA_Phase2 : Subsystem
  VIN : PMIOPort  Side=Left
  GND : PMIOPort  Port=2  Side=Left
  VOUT : PMIOPort  Port=3  Side=Right
  connections:
  VIN/RConn1 -- StageA_Phase1/LConn1 -- StageA_Phase2/LConn1
  GND/RConn1 -- StageA_Phase1/LConn2 -- StageA_Phase2/LConn2
  VOUT/RConn1 -- StageA_Phase1/RConn1 -- StageA_Phase2/RConn1

== system TB07_Integrated_Charging/StageA_Module2 ==
  note: Stage A 모듈 2: 위상 3·4 병렬(목표 정격 37.5 kW)
      | 각 위상은 영교차 추종 게이트로 자기 공진전류가 0일 때 끈다(ZCS). 두 위상은 T/4 엇갈려 시작한다.
  StageA_Phase3 : Subsystem
  StageA_Phase4 : Subsystem
  VIN : PMIOPort  Side=Left
  GND : PMIOPort  Port=2  Side=Left
  VOUT : PMIOPort  Port=3  Side=Right
  connections:
  VIN/RConn1 -- StageA_Phase3/LConn1 -- StageA_Phase4/LConn1
  GND/RConn1 -- StageA_Phase3/LConn2 -- StageA_Phase4/LConn2
  VOUT/RConn1 -- StageA_Phase3/RConn1 -- StageA_Phase4/RConn1

== system TB07_Integrated_Charging/StageA_Module3 ==
  note: Stage A 모듈 3: 위상 5·6 병렬(목표 정격 37.5 kW)
      | 각 위상은 영교차 추종 게이트로 자기 공진전류가 0일 때 끈다(ZCS). 두 위상은 T/4 엇갈려 시작한다.
  StageA_Phase5 : Subsystem
  StageA_Phase6 : Subsystem
  VIN : PMIOPort  Side=Left
  GND : PMIOPort  Port=2  Side=Left
  VOUT : PMIOPort  Port=3  Side=Right
  connections:
  VIN/RConn1 -- StageA_Phase5/LConn1 -- StageA_Phase6/LConn1
  GND/RConn1 -- StageA_Phase5/LConn2 -- StageA_Phase6/LConn2
  VOUT/RConn1 -- StageA_Phase5/RConn1 -- StageA_Phase6/RConn1

== system TB07_Integrated_Charging/StageA_Module4 ==
  note: Stage A 모듈 4: 위상 7·8 병렬(목표 정격 37.5 kW)
      | 각 위상은 영교차 추종 게이트로 자기 공진전류가 0일 때 끈다(ZCS). 두 위상은 T/4 엇갈려 시작한다.
  StageA_Phase7 : Subsystem
  StageA_Phase8 : Subsystem
  VIN : PMIOPort  Side=Left
  GND : PMIOPort  Port=2  Side=Left
  VOUT : PMIOPort  Port=3  Side=Right
  connections:
  VIN/RConn1 -- StageA_Phase7/LConn1 -- StageA_Phase8/LConn1
  GND/RConn1 -- StageA_Phase7/LConn2 -- StageA_Phase8/LConn2
  VOUT/RConn1 -- StageA_Phase7/RConn1 -- StageA_Phase8/RConn1

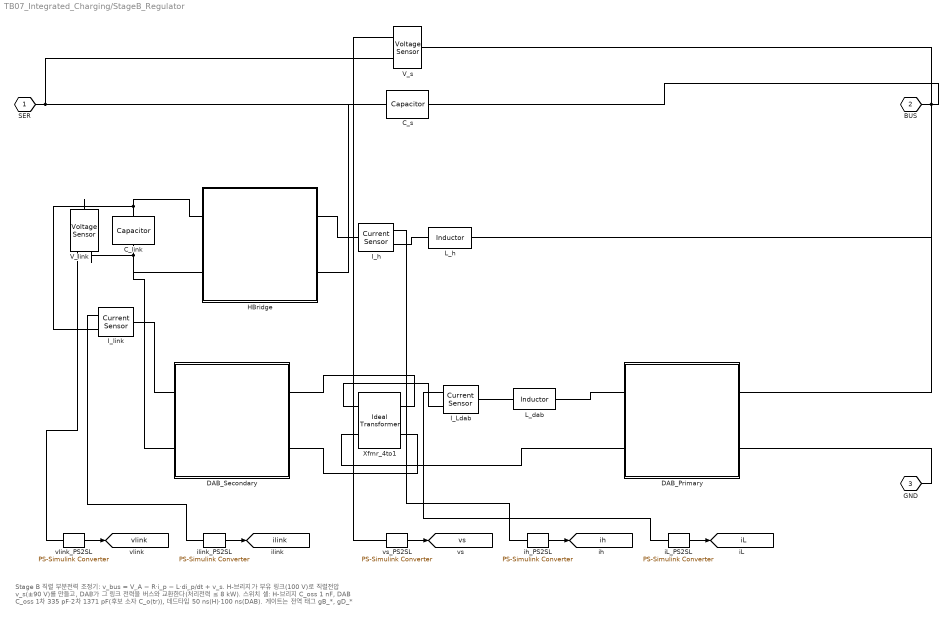
== system TB07_Integrated_Charging/StageB_Regulator ==
  note: Stage B 직렬 부분전력 조정기: v_bus = V_A − R·i_p − L·di_p/dt + v_s.
      | H-브리지가 부유 링크(100 V)로 직렬전압 v_s(±90 V)를 만들고, DAB가 그 링크 전력을 버스와 교환한다(처리전력 ≤ 8 kW).
      | 스위치 셀: H-브리지 C_oss 1 nF, DAB C_oss 1차 335 pF·2차 1371 pF(후보 소자 C_o(tr)), 데드타임 50 ns(H)·100 ns(DAB). 게이트는 전역 태그 gB_*, gD_*
  C_link : fl_lib/Electrical/Electrical Elements/Capacitor  c=TB.B.Clink F  r=1e-6 Ohm  g=0 1/Ohm  i_specify=off  i_priority=None  i=0 A  i_nominal_specify=off  i_nominal_value=1  i_nominal_unit=A  v_specify=off  v_priority=None  v=0 V  v_nominal_specify=off  v_nominal_value=1  v_nominal_unit=V  vc_specify=on  vc_priority=High  vc=TB.vl0 V  vc_nominal_specify=off  vc_nominal_value=1  vc_nominal_unit=V
  C_s : fl_lib/Electrical/Electrical Elements/Capacitor  c=TB.B.Cs F  r=1e-6 Ohm  g=0 1/Ohm  i_specify=off  i_priority=None  i=0 A  i_nominal_specify=off  i_nominal_value=1  i_nominal_unit=A  v_specify=off  v_priority=None  v=0 V  v_nominal_specify=off  v_nominal_value=1  v_nominal_unit=V  vc_specify=on  vc_priority=High  vc=TB.vs0 V  vc_nominal_specify=off  vc_nominal_value=1  vc_nominal_unit=V
  DAB_Primary : Subsystem
  DAB_Secondary : Subsystem
  HBridge : Subsystem
  I_Ldab : fl_lib/Electrical/Electrical Sensors/Current Sensor
  I_h : fl_lib/Electrical/Electrical Sensors/Current Sensor
  I_link : fl_lib/Electrical/Electrical Sensors/Current Sensor
  L_dab : fl_lib/Electrical/Electrical Elements/Inductor  l=TB.B.Ldab H  r=TB.B.Rdab Ohm  g=1e-9 1/Ohm  i_specify=off  i_priority=None  i=0 A  i_nominal_specify=off  i_nominal_value=1  i_nominal_unit=A  v_specify=off  v_priority=None  v=0 V  v_nominal_specify=off  v_nominal_value=1  v_nominal_unit=V  i_L_specify=on  i_L_priority=High  i_L=0 A  i_L_nominal_specify=off  i_L_nominal_value=1  i_L_nominal_unit=A
  L_h : fl_lib/Electrical/Electrical Elements/Inductor  l=TB.B.Lh H  r=TB.B.Rh Ohm  g=1e-9 1/Ohm  i_specify=off  i_priority=None  i=0 A  i_nominal_specify=off  i_nominal_value=1  i_nominal_unit=A  v_specify=off  v_priority=None  v=0 V  v_nominal_specify=off  v_nominal_value=1  v_nominal_unit=V  i_L_specify=on  i_L_priority=High  i_L=TB.ih0 A  i_L_nominal_specify=off  i_L_nominal_value=1  i_L_nominal_unit=A
  V_link : fl_lib/Electrical/Electrical Sensors/Voltage Sensor
  V_s : fl_lib/Electrical/Electrical Sensors/Voltage Sensor
  Xfmr_4to1 : fl_lib/Electrical/Electrical Elements/Ideal Transformer  n=TB.B.n  i1_specify=off  i1_priority=None  i1=0 A  i1_nominal_specify=off  i1_nominal_value=1  i1_nominal_unit=A  v1_specify=off  v1_priority=None  v1=0 V  v1_nominal_specify=off  v1_nominal_value=1  v1_nominal_unit=V  i2_specify=off  i2_priority=None  i2=0 A  i2_nominal_specify=off  i2_nominal_value=1  i2_nominal_unit=A  v2_specify=off  v2_priority=None  v2=0 V  v2_nominal_specify=off  v2_nominal_value=1  v2_nominal_unit=V
  iL_PS2SL : nesl_utility/PS-Simulink Converter  PhysicalDomain=network_engine_domain  SubClassName=ps_output  LeftPortType=input  RightPortType=output  PseudoPeriodic=off  Frequencies=[]  VectorFormat=inherit  Unit=inherit  AffineConversion=off
  ih_PS2SL : nesl_utility/PS-Simulink Converter  PhysicalDomain=network_engine_domain  SubClassName=ps_output  LeftPortType=input  RightPortType=output  PseudoPeriodic=off  Frequencies=[]  VectorFormat=inherit  Unit=inherit  AffineConversion=off
  ilink_PS2SL : nesl_utility/PS-Simulink Converter  PhysicalDomain=network_engine_domain  SubClassName=ps_output  LeftPortType=input  RightPortType=output  PseudoPeriodic=off  Frequencies=[]  VectorFormat=inherit  Unit=inherit  AffineConversion=off
  vlink_PS2SL : nesl_utility/PS-Simulink Converter  PhysicalDomain=network_engine_domain  SubClassName=ps_output  LeftPortType=input  RightPortType=output  PseudoPeriodic=off  Frequencies=[]  VectorFormat=inherit  Unit=inherit  AffineConversion=off
  vs_PS2SL : nesl_utility/PS-Simulink Converter  PhysicalDomain=network_engine_domain  SubClassName=ps_output  LeftPortType=input  RightPortType=output  PseudoPeriodic=off  Frequencies=[]  VectorFormat=inherit  Unit=inherit  AffineConversion=off
  SER : PMIOPort  Side=Left
  BUS : PMIOPort  Port=2  Side=Right
  GND : PMIOPort  Port=3  Side=Right
  tag scope: iL=global, ih=global, ilink=global, vlink=global, vs=global
  wires:
  vs_PS2SL/1 -> [vs]
  ih_PS2SL/1 -> [ih]
  vlink_PS2SL/1 -> [vlink]
  ilink_PS2SL/1 -> [ilink]
  iL_PS2SL/1 -> [iL]
  connections:
  C_s/RConn1 -- V_s/RConn2 -- SER/RConn1 -- HBridge/RConn2
  C_s/LConn1 -- V_s/LConn1 -- L_h/RConn1 -- BUS/RConn1 -- DAB_Primary/LConn1
  HBridge/RConn1 -- I_h/LConn1
  I_h/RConn2 -- L_h/LConn1
  HBridge/LConn1 -- C_link/LConn1 -- V_link/LConn1 -- I_link/RConn2
  HBridge/LConn2 -- C_link/RConn1 -- V_link/RConn2 -- DAB_Secondary/LConn2
  DAB_Secondary/LConn1 -- I_link/LConn1
  DAB_Secondary/RConn1 -- Xfmr_4to1/RConn1
  DAB_Secondary/RConn2 -- Xfmr_4to1/RConn2
  DAB_Primary/RConn1 -- L_dab/LConn1
  L_dab/RConn1 -- I_Ldab/LConn1
  I_Ldab/RConn2 -- Xfmr_4to1/LConn1
  Xfmr_4to1/LConn2 -- DAB_Primary/RConn2
  DAB_Primary/LConn2 -- GND/RConn1
  V_s/RConn1 -- vs_PS2SL/LConn1
  I_h/RConn1 -- ih_PS2SL/LConn1
  V_link/RConn1 -- vlink_PS2SL/LConn1
  I_link/RConn1 -- ilink_PS2SL/LConn1
  I_Ldab/RConn1 -- iL_PS2SL/LConn1

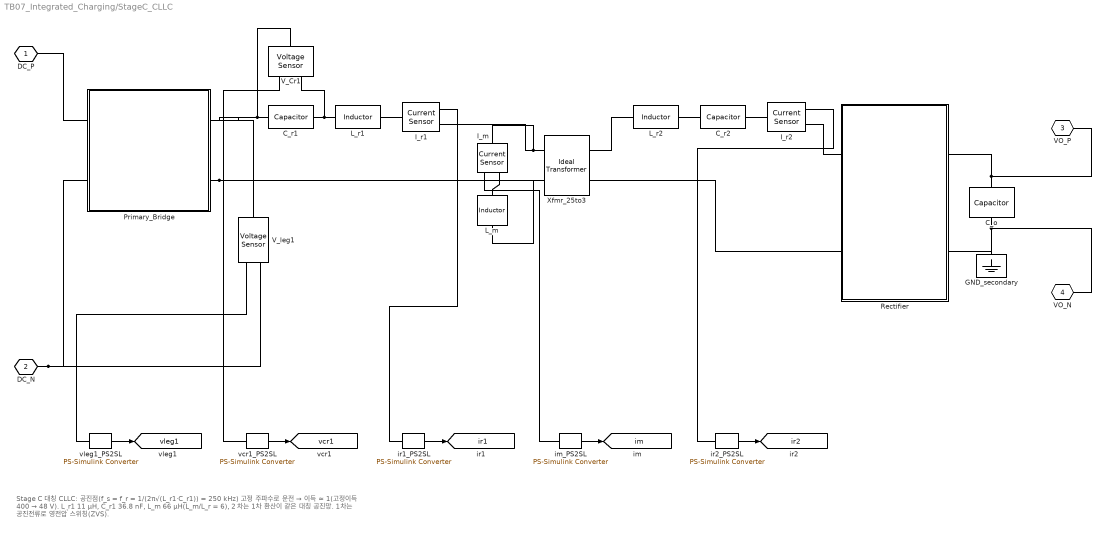
== system TB07_Integrated_Charging/StageC_CLLC ==
  note: Stage C 대칭 CLLC: 공진점(f_s = f_r = 1/(2π√(L_r1·C_r1)) = 250 kHz) 고정 주파수로 운전 → 이득 ≈ 1(고정이득 400 → 48 V).
      | L_r1 11 µH, C_r1 36.8 nF, L_m 66 µH(L_m/L_r = 6), 2차는 1차 환산이 같은 대칭 공진망. 1차는 공진전류로 영전압 스위칭(ZVS).
  C_o : fl_lib/Electrical/Electrical Elements/Capacitor  c=TB.C.Co F  r=1e-6 Ohm  g=0 1/Ohm  i_specify=off  i_priority=None  i=0 A  i_nominal_specify=off  i_nominal_value=1  i_nominal_unit=A  v_specify=off  v_priority=None  v=0 V  v_nominal_specify=off  v_nominal_value=1  v_nominal_unit=V  vc_specify=on  vc_priority=High  vc=TB.vo0 V  vc_nominal_specify=off  vc_nominal_value=1  vc_nominal_unit=V
  C_r1 : fl_lib/Electrical/Electrical Elements/Capacitor  c=TB.C.Cr1 F  r=1e-6 Ohm  g=0 1/Ohm  i_specify=off  i_priority=None  i=0 A  i_nominal_specify=off  i_nominal_value=1  i_nominal_unit=A  v_specify=off  v_priority=None  v=0 V  v_nominal_specify=off  v_nominal_value=1  v_nominal_unit=V  vc_specify=on  vc_priority=High  vc=0 V  vc_nominal_specify=off  vc_nominal_value=1  vc_nominal_unit=V
  C_r2 : fl_lib/Electrical/Electrical Elements/Capacitor  c=TB.C.Cr2 F  r=1e-6 Ohm  g=0 1/Ohm  i_specify=off  i_priority=None  i=0 A  i_nominal_specify=off  i_nominal_value=1  i_nominal_unit=A  v_specify=off  v_priority=None  v=0 V  v_nominal_specify=off  v_nominal_value=1  v_nominal_unit=V  vc_specify=on  vc_priority=High  vc=0 V  vc_nominal_specify=off  vc_nominal_value=1  vc_nominal_unit=V
  GND_secondary : fl_lib/Electrical/Electrical Elements/Electrical Reference
  I_m : fl_lib/Electrical/Electrical Sensors/Current Sensor
  I_r1 : fl_lib/Electrical/Electrical Sensors/Current Sensor
  I_r2 : fl_lib/Electrical/Electrical Sensors/Current Sensor
  L_m : fl_lib/Electrical/Electrical Elements/Inductor  l=TB.C.Lm H  r=0 Ohm  g=1e-9 1/Ohm  i_specify=off  i_priority=None  i=0 A  i_nominal_specify=off  i_nominal_value=1  i_nominal_unit=A  v_specify=off  v_priority=None  v=0 V  v_nominal_specify=off  v_nominal_value=1  v_nominal_unit=V  i_L_specify=on  i_L_priority=High  i_L=0 A  i_L_nominal_specify=off  i_L_nominal_value=1  i_L_nominal_unit=A
  L_r1 : fl_lib/Electrical/Electrical Elements/Inductor  l=TB.C.Lr1 H  r=0 Ohm  g=1e-9 1/Ohm  i_specify=off  i_priority=None  i=0 A  i_nominal_specify=off  i_nominal_value=1  i_nominal_unit=A  v_specify=off  v_priority=None  v=0 V  v_nominal_specify=off  v_nominal_value=1  v_nominal_unit=V  i_L_specify=on  i_L_priority=High  i_L=0 A  i_L_nominal_specify=off  i_L_nominal_value=1  i_L_nominal_unit=A
  L_r2 : fl_lib/Electrical/Electrical Elements/Inductor  l=TB.C.Lr2 H  r=0 Ohm  g=1e-9 1/Ohm  i_specify=off  i_priority=None  i=0 A  i_nominal_specify=off  i_nominal_value=1  i_nominal_unit=A  v_specify=off  v_priority=None  v=0 V  v_nominal_specify=off  v_nominal_value=1  v_nominal_unit=V  i_L_specify=on  i_L_priority=High  i_L=0 A  i_L_nominal_specify=off  i_L_nominal_value=1  i_L_nominal_unit=A
  Primary_Bridge : Subsystem
  Rectifier : Subsystem
  V_Cr1 : fl_lib/Electrical/Electrical Sensors/Voltage Sensor
  V_leg1 : fl_lib/Electrical/Electrical Sensors/Voltage Sensor
  Xfmr_25to3 : fl_lib/Electrical/Electrical Elements/Ideal Transformer  n=TB.C.n  i1_specify=off  i1_priority=None  i1=0 A  i1_nominal_specify=off  i1_nominal_value=1  i1_nominal_unit=A  v1_specify=off  v1_priority=None  v1=0 V  v1_nominal_specify=off  v1_nominal_value=1  v1_nominal_unit=V  i2_specify=off  i2_priority=None  i2=0 A  i2_nominal_specify=off  i2_nominal_value=1  i2_nominal_unit=A  v2_specify=off  v2_priority=None  v2=0 V  v2_nominal_specify=off  v2_nominal_value=1  v2_nominal_unit=V
  im_PS2SL : nesl_utility/PS-Simulink Converter  PhysicalDomain=network_engine_domain  SubClassName=ps_output  LeftPortType=input  RightPortType=output  PseudoPeriodic=off  Frequencies=[]  VectorFormat=inherit  Unit=inherit  AffineConversion=off
  ir1_PS2SL : nesl_utility/PS-Simulink Converter  PhysicalDomain=network_engine_domain  SubClassName=ps_output  LeftPortType=input  RightPortType=output  PseudoPeriodic=off  Frequencies=[]  VectorFormat=inherit  Unit=inherit  AffineConversion=off
  ir2_PS2SL : nesl_utility/PS-Simulink Converter  PhysicalDomain=network_engine_domain  SubClassName=ps_output  LeftPortType=input  RightPortType=output  PseudoPeriodic=off  Frequencies=[]  VectorFormat=inherit  Unit=inherit  AffineConversion=off
  vcr1_PS2SL : nesl_utility/PS-Simulink Converter  PhysicalDomain=network_engine_domain  SubClassName=ps_output  LeftPortType=input  RightPortType=output  PseudoPeriodic=off  Frequencies=[]  VectorFormat=inherit  Unit=inherit  AffineConversion=off
  vleg1_PS2SL : nesl_utility/PS-Simulink Converter  PhysicalDomain=network_engine_domain  SubClassName=ps_output  LeftPortType=input  RightPortType=output  PseudoPeriodic=off  Frequencies=[]  VectorFormat=inherit  Unit=inherit  AffineConversion=off
  DC_P : PMIOPort  Side=Left
  DC_N : PMIOPort  Port=2  Side=Left
  VO_P : PMIOPort  Port=3  Side=Right
  VO_N : PMIOPort  Port=4  Side=Right
  tag scope: im=global, ir1=global, ir2=global, vcr1=global, vleg1=global
  wires:
  ir1_PS2SL/1 -> [ir1]
  im_PS2SL/1 -> [im]
  ir2_PS2SL/1 -> [ir2]
  vcr1_PS2SL/1 -> [vcr1]
  vleg1_PS2SL/1 -> [vleg1]
  connections:
  Primary_Bridge/LConn1 -- DC_P/RConn1
  DC_N/RConn1 -- Primary_Bridge/LConn2 -- V_leg1/RConn2
  C_r1/LConn1 -- Primary_Bridge/RConn1 -- V_leg1/LConn1 -- V_Cr1/LConn1
  L_r1/LConn1 -- C_r1/RConn1 -- V_Cr1/RConn2
  L_r1/RConn1 -- I_r1/LConn1
  Xfmr_25to3/LConn1 -- I_r1/RConn2 -- I_m/LConn1
  Primary_Bridge/RConn2 -- Xfmr_25to3/LConn2 -- L_m/RConn1
  I_m/RConn2 -- L_m/LConn1
  Xfmr_25to3/RConn1 -- L_r2/LConn1
  L_r2/RConn1 -- C_r2/LConn1
  C_r2/RConn1 -- I_r2/LConn1
  I_r2/RConn2 -- Rectifier/LConn1
  Xfmr_25to3/RConn2 -- Rectifier/LConn2
  C_o/LConn1 -- Rectifier/RConn1 -- VO_P/RConn1
  Rectifier/RConn2 -- VO_N/RConn1 -- C_o/RConn1 -- GND_secondary/LConn1
  I_r1/RConn1 -- ir1_PS2SL/LConn1
  I_m/RConn1 -- im_PS2SL/LConn1
  I_r2/RConn1 -- ir2_PS2SL/LConn1
  V_Cr1/RConn1 -- vcr1_PS2SL/LConn1
  V_leg1/RConn1 -- vleg1_PS2SL/LConn1

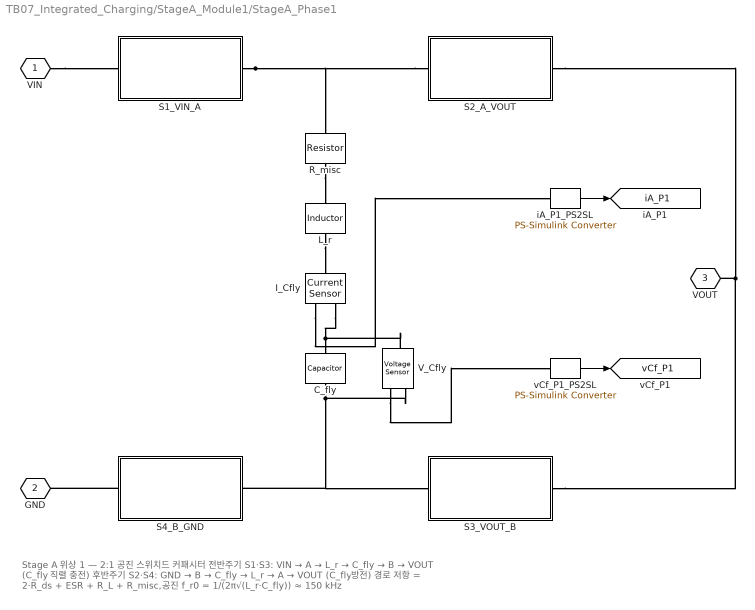
== system TB07_Integrated_Charging/StageA_Module1/StageA_Phase1 ==
  note: Stage A 위상 1 — 2:1 공진 스위치드 커패시터
      | 전반주기 S1·S3: VIN → A → L_r → C_fly → B → VOUT (C_fly 직렬 충전)
      | 후반주기 S2·S4: GND → B → C_fly → L_r → A → VOUT (C_fly 방전)
      | 경로 저항 = 2·R_ds + ESR + R_L + R_misc, 공진 f_r0 = 1/(2π√(L_r·C_fly)) ≈ 150 kHz
  C_fly : fl_lib/Electrical/Electrical Elements/Capacitor  c=TB.A.Cfly F  r=TB.A.ESR Ohm  g=0 1/Ohm  i_specify=off  i_priority=None  i=0 A  i_nominal_specify=off  i_nominal_value=1  i_nominal_unit=A  v_specify=off  v_priority=None  v=0 V  v_nominal_specify=off  v_nominal_value=1  v_nominal_unit=V  vc_specify=on  vc_priority=High  vc=TB.A.vC0 V  vc_nominal_specify=off  vc_nominal_value=1  vc_nominal_unit=V
  I_Cfly : fl_lib/Electrical/Electrical Sensors/Current Sensor
  L_r : fl_lib/Electrical/Electrical Elements/Inductor  l=TB.A.Lr H  r=TB.A.RL Ohm  g=1e-9 1/Ohm  i_specify=off  i_priority=None  i=0 A  i_nominal_specify=off  i_nominal_value=1  i_nominal_unit=A  v_specify=off  v_priority=None  v=0 V  v_nominal_specify=off  v_nominal_value=1  v_nominal_unit=V  i_L_specify=on  i_L_priority=High  i_L=0 A  i_L_nominal_specify=off  i_L_nominal_value=1  i_L_nominal_unit=A
  R_misc : fl_lib/Electrical/Electrical Elements/Resistor  R=TB.A.Rmisc Ohm  i_specify=off  i_priority=None  i=0 A  i_nominal_specify=off  i_nominal_value=1  i_nominal_unit=A  v_specify=off  v_priority=None  v=0 V  v_nominal_specify=off  v_nominal_value=1  v_nominal_unit=V
  S1_VIN_A : Subsystem  mask(PRISM-Hub switch cell){Ron=TB.A.Rds, Goff=TB.A.Goff, Vf=TB.A.Vf, Rd=TB.A.Rd, Goffd=TB.A.Goffd}
      mask prompts: Ron "도통 저항 R_on [Ohm]"; Goff "차단 컨덕턴스 G_off [S]"; Vf "다이오드 순방향 전압 Vf [V]"; Rd "다이오드 도통 저항 R_d [Ohm]"; Goffd "다이오드 차단 컨덕턴스 [S]"
      mask help: 전력 반도체 스위치 셀 S1. 게이트 태그 gA_P1_S1.
      settings: AttributesFormatString=gate: gA_P1_S1
      mask Display:
      | plot([0.05 0.35 ],[0.50 0.50 ],[0.35 0.65 ],[0.50 0.74 ],[0.65 0.95 ],[0.50 0.50 ]);
      | plot([0.20 0.20 0.42 ],[0.50 0.20 0.20 ],[0.58 0.80 0.80 ],[0.20 0.20 0.50 ]);
      | plot([0.42 0.58 0.58 0.42 ],[0.20 0.10 0.30 0.20 ],[0.42 0.42 ],[0.10 0.30 ]);
      | text(0.5,0.80,'S1','horizontalAlignment','center','texmode','off');
      | port_label('LConn',1,'D');
      | port_label('RConn',1,'S');
  S2_A_VOUT : Subsystem  mask(PRISM-Hub switch cell){Ron=TB.A.Rds, Goff=TB.A.Goff, Vf=TB.A.Vf, Rd=TB.A.Rd, Goffd=TB.A.Goffd}
      mask prompts: Ron "도통 저항 R_on [Ohm]"; Goff "차단 컨덕턴스 G_off [S]"; Vf "다이오드 순방향 전압 Vf [V]"; Rd "다이오드 도통 저항 R_d [Ohm]"; Goffd "다이오드 차단 컨덕턴스 [S]"
      mask help: 전력 반도체 스위치 셀 S2. 게이트 태그 gA_P1_S2.
      settings: AttributesFormatString=gate: gA_P1_S2
      mask Display:
      | plot([0.05 0.35 ],[0.50 0.50 ],[0.35 0.65 ],[0.50 0.74 ],[0.65 0.95 ],[0.50 0.50 ]);
      | plot([0.20 0.20 0.42 ],[0.50 0.20 0.20 ],[0.58 0.80 0.80 ],[0.20 0.20 0.50 ]);
      | plot([0.42 0.58 0.58 0.42 ],[0.20 0.10 0.30 0.20 ],[0.42 0.42 ],[0.10 0.30 ]);
      | text(0.5,0.80,'S2','horizontalAlignment','center','texmode','off');
      | port_label('LConn',1,'D');
      | port_label('RConn',1,'S');
  S3_VOUT_B : Subsystem  mask(PRISM-Hub switch cell){Ron=TB.A.Rds, Goff=TB.A.Goff, Vf=TB.A.Vf, Rd=TB.A.Rd, Goffd=TB.A.Goffd}
      mask prompts: Ron "도통 저항 R_on [Ohm]"; Goff "차단 컨덕턴스 G_off [S]"; Vf "다이오드 순방향 전압 Vf [V]"; Rd "다이오드 도통 저항 R_d [Ohm]"; Goffd "다이오드 차단 컨덕턴스 [S]"
      mask help: 전력 반도체 스위치 셀 S3. 게이트 태그 gA_P1_S3.
      settings: AttributesFormatString=gate: gA_P1_S3
      mask Display:
      | plot([0.95 0.65 ],[0.50 0.50 ],[0.65 0.35 ],[0.50 0.74 ],[0.35 0.05 ],[0.50 0.50 ]);
      | plot([0.80 0.80 0.58 ],[0.50 0.20 0.20 ],[0.42 0.20 0.20 ],[0.20 0.20 0.50 ]);
      | plot([0.58 0.42 0.42 0.58 ],[0.20 0.10 0.30 0.20 ],[0.58 0.58 ],[0.10 0.30 ]);
      | text(0.5,0.80,'S3','horizontalAlignment','center','texmode','off');
      | port_label('LConn',1,'D');
      | port_label('RConn',1,'S');
  S4_B_GND : Subsystem  mask(PRISM-Hub switch cell){Ron=TB.A.Rds, Goff=TB.A.Goff, Vf=TB.A.Vf, Rd=TB.A.Rd, Goffd=TB.A.Goffd}
      mask prompts: Ron "도통 저항 R_on [Ohm]"; Goff "차단 컨덕턴스 G_off [S]"; Vf "다이오드 순방향 전압 Vf [V]"; Rd "다이오드 도통 저항 R_d [Ohm]"; Goffd "다이오드 차단 컨덕턴스 [S]"
      mask help: 전력 반도체 스위치 셀 S4. 게이트 태그 gA_P1_S4.
      settings: AttributesFormatString=gate: gA_P1_S4
      mask Display:
      | plot([0.95 0.65 ],[0.50 0.50 ],[0.65 0.35 ],[0.50 0.74 ],[0.35 0.05 ],[0.50 0.50 ]);
      | plot([0.80 0.80 0.58 ],[0.50 0.20 0.20 ],[0.42 0.20 0.20 ],[0.20 0.20 0.50 ]);
      | plot([0.58 0.42 0.42 0.58 ],[0.20 0.10 0.30 0.20 ],[0.58 0.58 ],[0.10 0.30 ]);
      | text(0.5,0.80,'S4','horizontalAlignment','center','texmode','off');
      | port_label('LConn',1,'D');
      | port_label('RConn',1,'S');
  V_Cfly : fl_lib/Electrical/Electrical Sensors/Voltage Sensor
  iA_P1_PS2SL : nesl_utility/PS-Simulink Converter  PhysicalDomain=network_engine_domain  SubClassName=ps_output  LeftPortType=input  RightPortType=output  PseudoPeriodic=off  Frequencies=[]  VectorFormat=inherit  Unit=inherit  AffineConversion=off
  vCf_P1_PS2SL : nesl_utility/PS-Simulink Converter  PhysicalDomain=network_engine_domain  SubClassName=ps_output  LeftPortType=input  RightPortType=output  PseudoPeriodic=off  Frequencies=[]  VectorFormat=inherit  Unit=inherit  AffineConversion=off
  VIN : PMIOPort  Side=Left
  GND : PMIOPort  Port=2  Side=Left
  VOUT : PMIOPort  Port=3  Side=Right
  tag scope: iA_P1=global, vCf_P1=global
  wires:
  iA_P1_PS2SL/1 -> [iA_P1]
  vCf_P1_PS2SL/1 -> [vCf_P1]
  connections:
  VIN/RConn1 -- S1_VIN_A/LConn1
  S2_A_VOUT/LConn1 -- S1_VIN_A/RConn1 -- R_misc/LConn1
  R_misc/RConn1 -- L_r/LConn1
  L_r/RConn1 -- I_Cfly/LConn1
  C_fly/LConn1 -- I_Cfly/RConn2 -- V_Cfly/LConn1
  S4_B_GND/LConn1 -- C_fly/RConn1 -- S3_VOUT_B/RConn1 -- V_Cfly/RConn2
  S4_B_GND/RConn1 -- GND/RConn1
  VOUT/RConn1 -- S2_A_VOUT/RConn1 -- S3_VOUT_B/LConn1
  I_Cfly/RConn1 -- iA_P1_PS2SL/LConn1
  V_Cfly/RConn1 -- vCf_P1_PS2SL/LConn1
